simulink model "es_3_model_linear"  (R2024b)
settings: Solver=VariableStepAuto  StartTime=0.0  StopTime=T  RelTol=1e-3
libraries: robotmobilelib x1
settings Model: Creator=feder  LastModifiedBy=feder

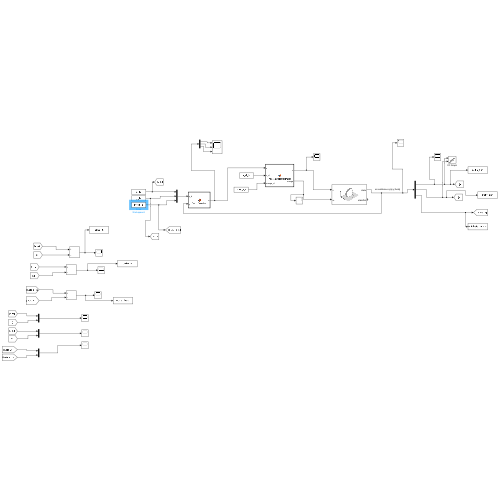
[thumbnail: Simulink's stored preview of the top-level diagram]
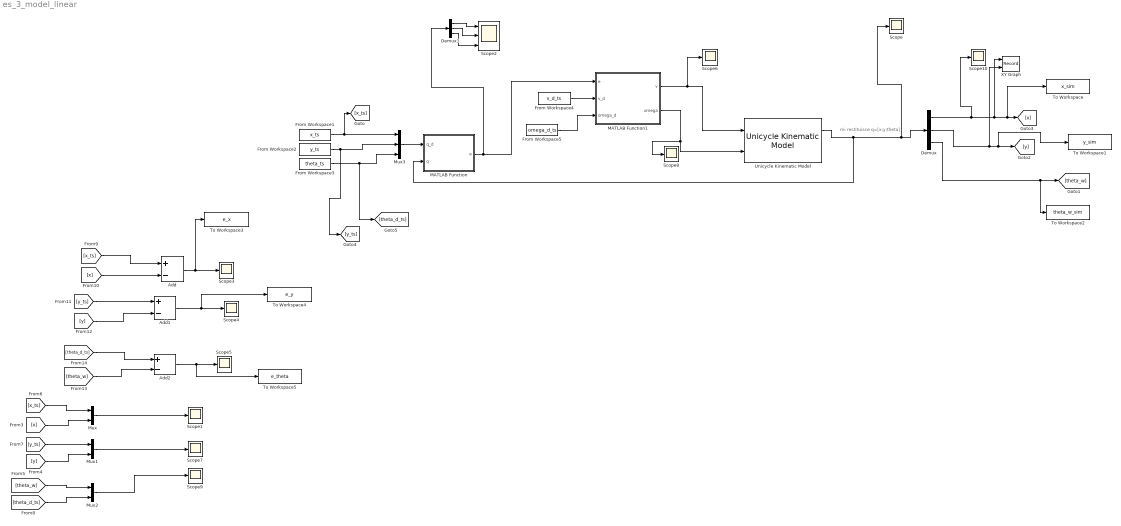
== system es_3_model_linear ==
  note: mi restituisce q=[x;y;theta]
  Add : Sum  Inputs=+-
  Add1 : Sum  Inputs=+-
  Add2 : Sum  Inputs=+-
  Demux : Demux  Outputs=3
  Demux1 : Demux  Outputs=3
  From Workspace1 : FromWorkspace  VariableName=x_ts
  From Workspace2 : FromWorkspace  VariableName=y_ts
  From Workspace3 : FromWorkspace  VariableName=theta_ts
  From Workspace4 : FromWorkspace  VariableName=v_d_ts
  From Workspace5 : FromWorkspace  VariableName=omega_d_ts
  MATLAB Function : MATLAB Function  TreatAsAtomicUnit=on
  MATLAB Function1 : MATLAB Function  TreatAsAtomicUnit=on
  Mux : Mux  Inputs=2
  Mux1 : Mux  Inputs=2
  Mux2 : Mux  Inputs=2
  Mux3 : Mux  Inputs=3
  Scope{,1,3..10} (10 alike) : Scope
  Scope2 : Scope  NumInputPorts=3
  To Workspace : ToWorkspace  VariableName=x_sim  SaveFormat=Timeseries  SampleTime=-1
  To Workspace1 : ToWorkspace  VariableName=y_sim  SaveFormat=Timeseries  SampleTime=-1
  To Workspace2 : ToWorkspace  VariableName=theta_w_sim  SaveFormat=Timeseries  SampleTime=-1
  To Workspace3 : ToWorkspace  VariableName=e_x  SaveFormat=Timeseries  SampleTime=-1
  To Workspace4 : ToWorkspace  VariableName=e_y  SaveFormat=Timeseries  SampleTime=-1
  To Workspace5 : ToWorkspace  VariableName=e_theta  SaveFormat=Timeseries  SampleTime=-1
  Unicycle Kinematic Model : robotmobilelib/Unicycle Kinematic Model  VehicleInputs=Vehicle Speed & Heading Angular Velocity  WheelRadius=0.1  WheelSpeedRange=[-Inf Inf]  InitialState=initial_state  SimulateUsing=Interpreted execution
  XY Graph : Record  FileSettingsInternal="{\"entries\":[{\"content\":{\"excelSettings\":{\"content\":{},\"type\":\"Streamout.ExcelSettings\"}},\"type\":\"Streamout.FileSettingStorage\",\"uuid\":\"\"}],\"packageUris\":[\"http:\\/\\/schema.mathworks.com\\/mf0\\/streamout_blocks\\/R2020a\"],\"version\":\"1.0\"}"  Layout=[1 1]  SignalsInternal="{\"entries\":[{\"content\":{\"signals\":[{\"content\":{\"blockPath\":[],\"dimensions\":[1],\"domain\":\"\",\"lineColor\":\"#a2142f\",\"plots\":[ 1 ],\"port\":1,\"sid\":[\"\"],\"signalID\":1,\"signalName\":\"Demux:1\"},\"type\":\"RecordBlkView.Signal\",\"uuid\":\"\"},{\"content\":{\"blockPath\":[],\"dimensions\":[1],\"domain\":\"\",\"lineColor\":\"#139fff\",\"plots\":[ 1 ],\"port\":2,\"sid\":[\"\"],\"signalID\":2,\"signalName\":\"Demux:2\"},\"type\":\"RecordBlkView.Signal\",\"uuid\":\"\"}]},\"type\":\"RecordBlkView.InputSignals\",\"uuid\":\"\"}],\"packageUris\":[\"http:\\/\\/schema.mathworks.com\\/mf0\\/streamout_blocks\\/R2020a\"],\"version\":\"1.0\"}"  VisualizationBindings="{\"xyplotplugin\":{\"info\":[{\"series\":[{\"bindingParametersList\":[{\"parameter\":\"X-Axis\",\"signalID\":1,\"signalName\":\"Demux:1\"},{\"parameter\":\"Y-Axis\",\"signalID\":2,\"signalName\":\"Demux:2\"}],\"seriesID\":0}],\"subplotID\":1}]}}"  CompatibilityTag=XY
  wires:
  [theta_d_ts] -> Add2/1
  [y] -> Mux1/2
  [x_ts] -> Mux/1
  [x_ts] -> Add/1
  [x] -> Add/2
  [y_ts] -> Add1/1
  Mux/1 -> Scope1/1
  Demux/2 -> XY Graph/2, To Workspace1/1, [y]
  Demux/1 -> Scope10/1, XY Graph/1, To Workspace/1, [x]
  Add2/1 -> To Workspace5/1, Scope5/1
  Mux1/1 -> Scope7/1
  Add1/1 -> To Workspace4/1, Scope4/1
  Add/1 -> To Workspace3/1, Scope3/1
  Mux2/1 -> Scope9/1
  [theta_d_ts] -> Mux2/2
  [y_ts] -> Mux1/1
  [x] -> Mux/2
  [theta_w] -> Add2/2
  [y] -> Add1/2
  [theta_w] -> Mux2/1
  Unicycle Kinematic Model/1 -> MATLAB Function/2(q), Scope/1, Demux/1
  From Workspace1/1 -> [x_ts], Mux3/1
  From Workspace2/1 -> [y_ts], Mux3/2
  From Workspace3/1 -> [theta_d_ts], Mux3/3
  Mux3/1 -> MATLAB Function/1(q_d)
  MATLAB Function/1(e) -> Demux1/1, MATLAB Function1/1(e)
  From Workspace4/1 -> MATLAB Function1/2(v_d)
  From Workspace5/1 -> MATLAB Function1/3(omega_d)
  MATLAB Function1/1(v) -> Scope6/1, Unicycle Kinematic Model/1
  MATLAB Function1/2(omega) -> Scope8/1, Unicycle Kinematic Model/2
  Demux1/1 -> Scope2/1
  Demux1/2 -> Scope2/2
  Demux1/3 -> Scope2/3
  Demux/3 -> To Workspace2/1, [theta_w]

== matlab function es_3_model_linear/MATLAB Function1 ==
  data: e input; v output; v_d input; omega_d input; omega output
function [v, omega] = ApproximateController(e, v_d, omega_d)

a= 200;      
zeta = 0.9;       
k1 = 2 * zeta * a;
k3 = 2 * zeta * a;

% Calcolo di k2(t)
if abs(v_d) > 1e-3
    k2 = (a^2 - omega_d) / v_d;
else
    k2 = 0; 
end

e1 = e(1);
e2 = e(2);
e3 = e(3);

u1 = -k1 * e1;
u2 = -k2 * e2 - k3 * e3;

v = v_d * cos(e3) - u1;
omega = omega_d - u2;
end

== matlab function es_3_model_linear/MATLAB Function ==
  data: q_d input; e output; q input
function e = Error_Rotation(q_d, q)
% Calcolo dell'errore nello stato per approximate linearization

% Ingressi:
% q_d = [x_d; y_d; theta_d]   → stato desiderato
% q   = [x;   y;   theta]     → stato attuale

% Output:
% e = [e1; e2; e3] = errore ruotato nel frame del robot

% Estrazione
x_d = q_d(1);
y_d = q_d(2);
theta_d = q_d(3);

x = q(1);
y = q(2);
theta = q(3);

% Differenza tra gli stati
delta = [x_d - x; y_d - y; theta_d - theta];

% Wrappa l'errore angolare in [-pi, pi]
%delta(3) = atan2(sin(delta(3)), cos(delta(3)));

% Rotazione inversa R^T(theta)
R = [ cos(theta),  sin(theta), 0;
     -sin(theta),  cos(theta), 0;
      0,           0,          1];

% Errore ruotato nel frame del robot
e = R * delta;
end
